simulink model "pd_control_qs3"  (R2026a)
settings: Solver=ode1  StopTime=9.99  FixedStep=0.002  AbsTol=1e-6  EnableMultiTasking=on
undefined symbols (not defined in the file or in its folder): HIL, qc_get_step_size
libraries: quarc_library x4, simulink x2
settings Model: SimulationMode=external  ExtModeTrigDuration=5000  Creator=MLevis  LastModifiedBy=User
settings SolverCC: PositivePriorityOrder=on
settings DataIOCC: SignalLoggingSaveFormat=ModelDataLogs
settings OptimizationCC: BooleanDataType=off  OptimizeBlockIOStorage=off  BufferReuse=off  GlobalBufferReuse=off  ExpressionFolding=off  LocalBlockOutputs=off  InitFltsAndDblsToZero=on  OptimizeDataStoreBuffers=off  BusAssignmentInplaceUpdate=off
settings DebuggingCC: SaveWithParameterizedLinksMsg=none  UnderspecifiedInitializationDetection=Classic  SignalResolutionControl=TryResolveAllWithWarning  MultiTaskDSMMsg=warning  MultiTaskCondExecSysMsg=none
settings HardwareCC: TargetHWDeviceType=32-bit Generic
settings RTWCC: SystemTargetFile=quarc_win64.tlc  TemplateMakefile=quarc_default_tmf  Toolchain=QUARC win64 | nmake (64-bit Windows)  BuildConfiguration=Faster Runs  Description=QUARC Win64 Target Using Toolchain
settings STFCustomTargetCC: SystemTargetFile=quarc_win64.tlc  MultiwordLength=2048.0  ConcurrentExecutionCompliant=on  UseToolchainInfoCompliant=on
settings GRTTargetCC: ExtMode=on  ExtModeMexFile=quarc_comm  ParMdlRefBuildCompliant=off  CompOptLevelCompliant=off  CombineOutputUpdateFcns=off  MatFileLogging=off  CPPClassGenCompliant=off  GRTInterface=on

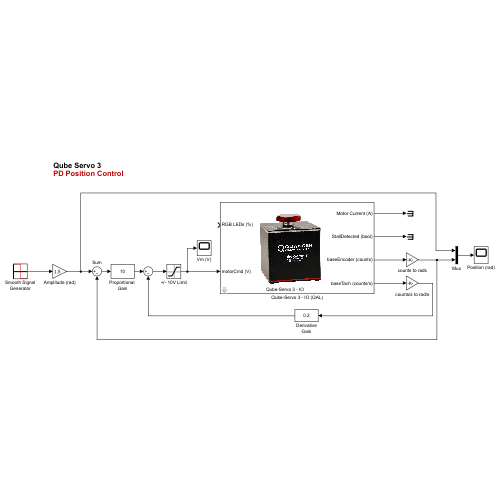
[thumbnail: Simulink's stored preview of the top-level diagram]
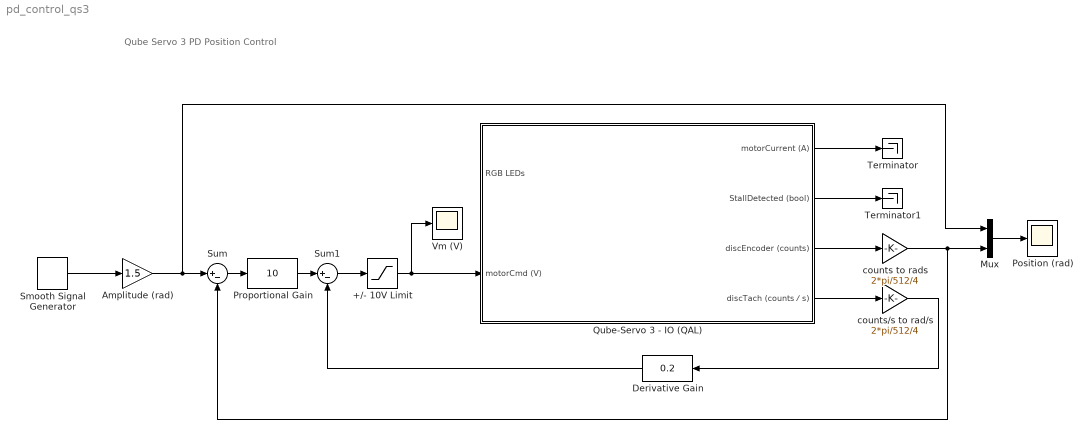
== system pd_control_qs3 ==
  note: Qube Servo 3
      | PD Position Control
  +/- 10V Limit : Saturate  UpperLimit=10  LowerLimit=-10
  Amplitude (rad) : Gain  Gain=1.5
  Derivative Gain : simulink/Math Operations/Slider Gain  gain=0.2  low=0  high=0.5
  Mux : Mux  Inputs=2
  Position (rad) : Scope
      settings: ActiveDisplayYMinimum=-1.8607039043124529  ActiveDisplayYMaximum=1.8937140740376548  DataLoggingSaveFormat=Array
  Proportional Gain : simulink/Math Operations/Slider Gain  gain=10  low=0  high=10
  Qube-Servo 3 - IO (QAL) : Subsystem  mask{setup=Hardware, top=Disc, QubeID=0}
      mask prompts: setup "Qube-Servo Setup:"; top "Qube Add-On:"; QubeID "Qube-Servo 3 Device Number:"
      mask help:
      | This subsystem provides the core and basic I/O capabilities to read data from and write data to the Qube-Servo 3 using the Quanser HIL API. You can write motor commands and LEDs and read motor current, motor stall detection, and base and pendulum encoder and tachometer.
      |
      | The RGB LEDs command is a 3x1 vector representing,
      | 1. Red LED
      | 2. Green LED
      | 3. Blue LED
      mask init:
      | % Initialization code section
      |     % HIL INITIALIZE OPTIONS
      |     % make sure hil initialize has the boardnumber we just created, will
      |     % get overwritten if virtual qube
      |     QubeNumber = get_param(gcb, 'QubeID');
      |     
      |     % Set up QubeID ip and portnumber in the hil initialize. 
      |     if strcmp(get_param(gcb, 'setup'), 'Hardware')
      |         set_param([gcb, '/HIL Initialize'], 'board_number', QubeNumber);
      |     elseif strcmp(get_param(gcb, 'setup'), 'Virtual') && strcmp(get_param(gcb, 'top'), 'Disc')
      |         set_param([gcb, '/HIL Initialize'], 'board_number', '0@tcpip://localhost:18922');
      |         
      |     elseif strcmp(get_param(gcb, 'setup'), 'Virtual') && strcmp(get_param(gcb, 'top'), 'Pendulum')
      |         set_param([gcb, '/HIL Initialize'], 'board_number', '0@tcpip://localhost:18923');
      |     end
      | 
      |     % make sure board specific options for qube are always set
      |     set_param([gcb, '/HIL Initialize'], 'board_options', 'deadband_compensation=0.3;pwm_en=0;enc0_velocity=3.0;enc1_velocity=3.0;min_diode_compensation=0.3;max_diode_compensation=1.5');
      |     
      |     % Delete 4 existing outport lines and if the other 2 exist, also delete
      |     location = get_param([gcb,'/motorCurrent (A)'],'PortConnectivity').Position;
      |     delete_line(gcbh,location);
      | 
      |     location = get_param([gcb,'/discEncoder (counts)'],'PortConnectivity').Position;
      |     delete_line(gcbh,location);
      | 
      |     location = get_param([gcb,'/StallDetected (bool)'],'PortConnectivity').Position;
      |     delete_line(gcbh,location);
      | 
      |     location = get_param([gcb,'/discTach (counts／s)'],'PortConnectivity').Position;
      |     delete_line(gcbh,location);
      | 
      |     pendulum_encoder_name = 'pendulumEncoder (counts)';
      |     pendulum_encoder = [gcb,'/',pendulum_encoder_name];
      | 
      |     pendulum_tach_name = 'pendulumTach (counts／s)';
      |     pendulum_tach = [gcb,'/',pendulum_tach_name];
      | 
      |     if ~isempty(find_system(gcbh,'LookUnderMasks','all','Name',pendulum_encoder_name))
      |        location = get_param(pendulum_encoder,'PortConnectivity').Position;
      |        delete_line(gcbh,location);
      |        delete_block(pendulum_encoder);
      |     end
      |     if ~isempty(find_system(gcbh,'LookUnderMasks','all','Name',pendulum_tach_name))
      |         location = get_param(pendulum_tach,'PortConnectivity').Position;
      |         delete_line(gcbh,location);
      |         delete_block(pendulum_tach);
      |     end
      | 
      |     % swap betweeen timebase or hil read
      |     timebase_name = 'HIL Read Timebase';
      | 
      |     read_name = 'HIL Read';
      |     
      |     if strcmp(QubeNumber, '0') % delete hil read if it exists and swap for timebase
      |         readBlock_name = timebase_name;
      |         readBlock = [gcb,'/',readBlock_name];
      |         if ~isempty(find_system(gcbh,'LookUnderMasks','all','Name',read_name))
      |             delete_block([gcb,'/',read_name]);
      |         end
      |         if isempty(find_system(gcbh,'LookUnderMasks','all','Name',timebase_name))
      |             add_block('quarc_library/Data Acquisition/Generic/Timebases/HIL Read Timebase',readBlock,'Position',[755,381,845,669]);
      |         end
      |         
      |     else % delete timebase if it exists, and change for hil read
      |         readBlock_name = read_name;
      |         readBlock = [gcb,'/',readBlock_name];
      |         if ~isempty(find_system(gcbh,'LookUnderMasks','all','Name',timebase_name))
      |             delete_block([gcb,'/',timebase_name]);
      |         end
      |         if isempty(find_system(gcbh,'LookUnderMasks','all','Name',read_name))
      |             add_block('quarc_library/Data Acquisition/Generic/Immediate I//O/HIL Read',readBlock,'Position',[755,381,845,669]);
      |         end
      |     end
      | 
      |     % make sure hil blocks match the hil initialize name
      |     set_param([gcb, '/HIL Write'], 'object_name', get_param([gcb, '/HIL Initialize'], 'object_name'));
      |     set_param(readBlock, 'object_name', get_param([gcb, '/HIL Initialize'], 'object_name'));
      | 
      |     % if nothing is connected to LED, we read RED which will always be 0 so
      |     % that the qube can turn green okay. Once something is connected, we
      |     % read all rgb channels
      |     blockPortData=get_param(gcb,'PortConnectivity');
      |     if (blockPortData(1).SrcBlock==-1)
      |         set_param([gcb, '/HIL Write'], 'other_channels', '[11000]');
      |     else
      |         set_param([gcb, '/HIL Write'], 'other_channels', '[11000:11002]');
      |     end
      | 
      |     % configure hil read outports to read everything
      |     set_param(readBlock, 'analog_channels', '[0]');
      |     set_param(readBlock, 'encoder_channels', '[0:1]');
      |     set_param(readBlock, 'digital_channels', '[1]');
      |     set_param(readBlock, 'other_channels', '[14000:14001]');
      | 
      |     % % if HIL read timebase, set up advanced settings
      |     if strcmp(readBlock_name, timebase_name)
      |         if strcmp(get_param(gcb, 'setup'), 'Hardware')
      |             set_param(readBlock, 'overflow_mode', 'Error on overflow');
      |             set_param(readBlock, 'samples_in_buffer', 'max(ceil(1/qc_get_step_size), 1)'); 
      |         else % virtual
      |             set_param(readBlock, 'overflow_mode', 'Synchronize (for simulated cards only)');
      |             set_param(readBlock, 'samples_in_buffer', '1');
      |         end
      |     end
      | 
      |     % connect all outports depending on read timebase or normal read
      |     add_line(gcbh,[readBlock_name,'/1'],['motorCurrent (A)','/1'],'autorouting','on');
      |     add_line(gcbh,[readBlock_name,'/2'],['discEncoder (counts)','/1'],'autorouting','on');
      |     add_line(gcbh,[readBlock_name,'/4'],['StallDetected (bool)','/1'],'autorouting','on');
      |     add_line(gcbh,[readBlock_name,'/5'],['discTach (counts／s)','/1'],'autorouting','on');
      | 
      | 
      |     % create pendulum encoder and pendulum tach ports and connections if
      |     % needed. Delete them if using the disc.
      |     if strcmp(get_param(gcb, 'top'), 'Pendulum')
      |         if isempty(find_system(gcbh,'LookUnderMasks','all','Name',pendulum_encoder_name))
      |             add_block('built-in/Outport',pendulum_encoder, 'Port','5','Position',[1050,568,1080,582]);
      |             add_line(gcbh,[readBlock_name,'/3'],[pendulum_encoder_name,'/1'],'autorouting','on');
      |         end
      |         if isempty(find_system(gcbh,'LookUnderMasks','all','Name',pendulum_tach_name))
      |             add_block('built-in/Outport',pendulum_tach, 'Port','6','Position',[1050, 603, 1080,617]);
      |             add_line(gcbh,[readBlock_name,'/6'],[pendulum_tach_name,'/1'],'autorouting','on');
      |         end 
      |     end
      | 
      |     % if virtual disc, only read pendulum tach. Take off pendulum tach from
      |     % options
      |     if strcmp(get_param(gcb, 'setup'), 'Virtual') && strcmp(get_param(gcb, 'top'), 'Disc')
      |         set_param(readBlock, 'other_channels', '[14000]');
      |     end
      settings: CopyFcn=set_param(gcbh,'LinkStatus','none');
      mask TypeOptions setup: Hardware | Virtual
      mask TypeOptions top: Disc | Pendulum
      mask TypeOptions QubeID: 0 | 1 | 2 | 3
      mask DialogControl AdvParameterGroupVar Prompt: Advanced Parameters (Multiple Qube-Servo 3's)
      mask DialogControl Control2 Prompt: Change this parameter when attempting to use more than one Qube-Servo 3. Assign different device numbers for different Qube-Servo 3's in ascending order starting with 0. If using one physical and one virtual in the same model, the physical one needs to be device number 0.
      mask Display:
      | ud = get_param(gcb,'UserData');
      | if (strcmp(get_param(gcb, 'top'), 'Disc') && strcmp(get_param(gcb, 'setup'), 'Hardware'))
      |     image(ud.hardwareDisc);
      | elseif (strcmp(get_param(gcb, 'top'), 'Pendulum') && strcmp(get_param(gcb, 'setup'), 'Hardware'))
      |     image(ud.hardwarePendulum);
      | elseif (strcmp(get_param(gcb, 'top'), 'Disc') && strcmp(get_param(gcb, 'setup'), 'Virtual'))
      |     image(ud.virtualDisc);
      | else
      |     image(ud.virtualPendulum);
      | end
      | 
      | text(.3,.05,'Qube-Servo 3 - IO');
      | 
      | if strcmp(get_param(gcb, 'top'), 'Pendulum')
      |     port_label('input', 1, 'RGB LEDs (%)');
      |     port_label('input', 2, 'motorCmd (V)');
      |     port_label('output', 1, 'Motor Current (A)');
      |     port_label('output', 2, 'StallDetected (bool)');
      |     port_label('output', 3, 'baseEncoder (counts)');
      |     port_label('output', 4, 'baseTach (counts/s)');
      |     port_label('output', 5, 'pendulumEncoder (counts)');
      |     port_label('output', 6, 'pendulumTach (counts/s)');
      | 
      | else
      |     port_label('input', 1, 'RGB LEDs (%)');
      |     port_label('input', 2, 'motorCmd (V)');
      |     port_label('output', 1, 'Motor Current (A)');
      |     port_label('output', 2, 'StallDetected (bool)');
      |     port_label('output', 3, 'baseEncoder (counts)');
      |     port_label('output', 4, 'baseTach (counts/s)');
      | end
  Smooth Signal Generator : quarc_library/Sources/Signals/Smooth Signal Generator  signal_type=Square  source=Internal (dialog parameters)  amplitude=1  frequency=0.4  initial_phase=0  sample_time=qc_get_step_size  output_cos=off
      settings: SourceProductName=QUARC Targets
  Sum : Sum  Inputs=|+-
  Sum1 : Sum  Inputs=|+-
  Terminator : Terminator
  Terminator1 : Terminator
  Vm (V) : Scope
      settings: ActiveDisplayYMinimum=-13.203683035714281  ActiveDisplayYMaximum=15.736941964285727  DataLoggingSaveFormat=Array
  counts to rads : Gain  Gain=2*pi/512/4
  counts/s to rad/s : Gain  Gain=2*pi/512/4
  wires:
  counts/s to rad/s/1 -> Derivative Gain/1
  Derivative Gain/1 -> Sum1/2
  Qube-Servo 3 - IO (QAL)/4(discTach (counts／s)) -> counts/s to rad/s/1
  Sum1/1 -> +/- 10V Limit/1
  Proportional Gain/1 -> Sum1/1
  Amplitude (rad)/1 -> Mux/1, Sum/1
  counts to rads/1 -> Mux/2, Sum/2
  Qube-Servo 3 - IO (QAL)/2(StallDetected (bool)) -> Terminator1/1
  Qube-Servo 3 - IO (QAL)/1(motorCurrent (A)) -> Terminator/1
  Qube-Servo 3 - IO (QAL)/3(discEncoder (counts)) -> counts to rads/1
  Mux/1 -> Position (rad)/1
  Sum/1 -> Proportional Gain/1
  Smooth Signal Generator/1 -> Amplitude (rad)/1
  +/- 10V Limit/1 -> Qube-Servo 3 - IO (QAL)/2(motorCmd (V)), Vm (V)/1

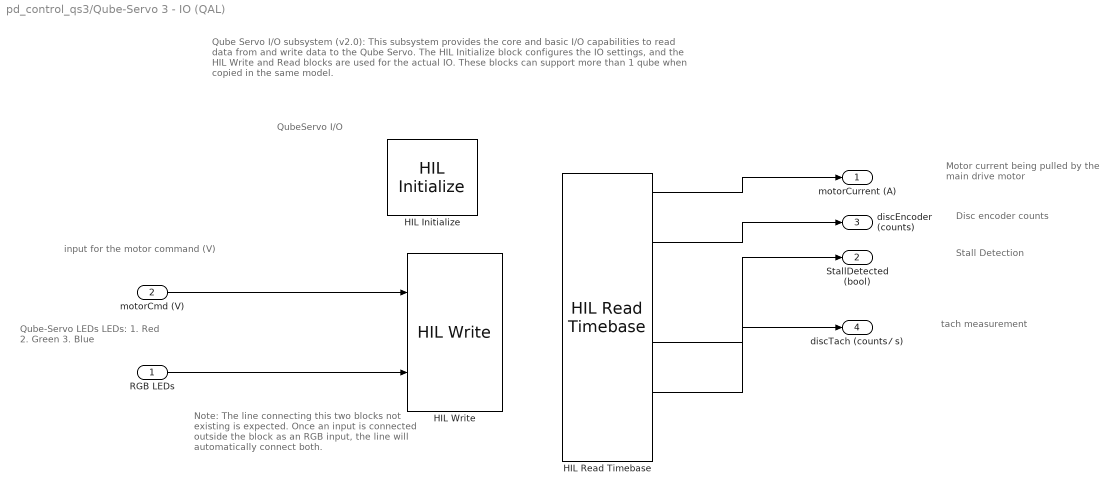
== system pd_control_qs3/Qube-Servo 3 - IO (QAL) ==
  note: Motor current being pulled by the main drive motor
  note: Stall Detection
  note: tach measurement
  note: Disc encoder counts
  note: input for the motor command (V)
  note: Qube Servo I/O subsystem (v2.0):
      |
      | This subsystem provides the core and basic I/O capabilities to read data from and write data to the Qube Servo. The HIL Initialize block configures the IO settings, and the HIL Write and Read blocks are used for the actual IO. These blocks can support more than 1 qube when copied in the same model.
  note: QubeServo I/O
  note: Qube-Servo LEDs
      |
      | LEDs:
      | 1. Red
      | 2. Green
      | 3. Blue
  note: Note: The line connecting this two blocks
      | not existing is expected.
      | Once an input is connected outside the block
      | as an RGB input, the line will automatically
      | connect both.
  RGB LEDs : Inport
  motorCmd (V) : Inport  Port=2
  HIL Initialize : quarc_library/Data Acquisition/Generic/Configuration/HIL Initialize  object_name=HIL-1  board_type=qube_servo3_usb  board_number=0  board_options=deadband_compensation=0.3;pwm_en=0;enc0_velocity=3.0;enc1_velocity=3.0;min_diode_compensation=0.3;max_diode_compensation=1.5  exclusive=off  active=on  hardware_clocks=[0]  clock_modes=[]  initial_clock_frequencies=[]  set_clock_params_at_start=off  set_clock_params_at_switch_in=off  set_clock_frequencies_at_start=off  set_clock_frequencies_at_switch_in=off  analog_input_channels=[0]  analog_input_configurations=[]  analog_input_maximums=3  analog_input_minimums=-3  set_analog_input_params_at_start=off  set_analog_input_params_at_switch_in=off  analog_output_channels=[0]  analog_output_maximums=15  analog_output_minimums=-15  initial_analog_outputs=[0]  final_analog_outputs=[0]  watchdog_analog_outputs=0  set_analog_output_params_at_start=off  set_analog_output_params_at_switch_in=off  set_analog_outputs_at_start=on  set_analog_outputs_at_switch_in=off  set_analog_outputs_at_terminate=on  set_analog_outputs_at_switch_out=off  set_analog_outputs_on_watchdog=on  digital_input_channels=[]  digital_output_channels=[0]  digital_output_configuration=[]  initial_digital_outputs=[1]  final_digital_outputs=[0]  watchdog_digital_outputs=[0]  set_digital_output_params_at_start=off  set_digital_output_params_at_switch_in=off  set_digital_outputs_at_start=on  set_digital_outputs_at_switch_in=off  set_digital_outputs_at_terminate=on  set_digital_outputs_at_switch_out=off  set_digital_outputs_on_watchdog=on  encoder_channels=[0:1]  quadrature=[4]  encoder_filter_frequency=[]  initial_encoder_counts=[0]  set_encoder_params_at_start=off  set_encoder_params_at_switch_in=off  set_encoder_counts_at_start=on  set_encoder_counts_at_switch_in=off  pwm_channels=[]  pwm_modes=[0]  pwm_frequency=23195  pwm_configuration=[1]  pwm_alignment=[0]  pwm_polarity=[1]  pwm_leading_deadband=[0]  pwm_trailing_deadband=[0]  initial_pwm_outputs=[0]  final_pwm_outputs=[0]  watchdog_pwm_outputs=[]  set_pwm_params_at_start=off  set_pwm_params_at_switch_in=off  set_pwm_outputs_at_start=off  set_pwm_outputs_at_switch_in=off  set_pwm_outputs_at_terminate=off  set_pwm_outputs_at_switch_out=off  set_pwm_outputs_on_watchdog=off  other_output_channels=[11000:11002]  initial_other_outputs=[0 1 0]  final_other_outputs=[1 0 0]  watchdog_other_outputs=[0 0 1]  set_other_outputs_at_start=on  set_other_outputs_at_switch_in=off  set_other_outputs_at_terminate=on  set_other_outputs_at_switch_out=off  set_other_outputs_on_watchdog=on
  HIL Read Timebase : quarc_library/Data Acquisition/Generic/Timebases/HIL Read Timebase  object_name=HIL-1  clock=0  analog_channels=[0]  encoder_channels=[0:1]  digital_channels=[1]  other_channels=[14000:14001]  active=on  vector_output=off  port_labels=channel numbers  data_type_mode=Inherit via back propagation  encoder_data_type=double  digital_data_type=boolean  overflow_mode=Error on overflow  samples_in_buffer=max(ceil(1/qc_get_step_size), 1)
  HIL Write : quarc_library/Data Acquisition/Generic/Immediate I//O/HIL Write  object_name=HIL-1  analog_channels=[0]  pwm_channels=[]  digital_channels=[]  other_channels=[11000]  sample_time=-1  active=off  vector_input=off  port_labels=channel numbers
  motorCurrent (A) : Outport  VectorParamsAs1DForOutWhenUnconnected=off
  StallDetected (bool) : Outport  Port=2  VectorParamsAs1DForOutWhenUnconnected=off
  discEncoder (counts) : Outport  Port=3  VectorParamsAs1DForOutWhenUnconnected=off
  discTach (counts／s) : Outport  Port=4  VectorParamsAs1DForOutWhenUnconnected=off
  wires:
  RGB LEDs/1 -> HIL Write/2
  motorCmd (V)/1 -> HIL Write/1
  HIL Read Timebase/1 -> motorCurrent (A)/1
  HIL Read Timebase/2 -> discEncoder (counts)/1
  HIL Read Timebase/4 -> StallDetected (bool)/1
  HIL Read Timebase/5 -> discTach (counts／s)/1
